simulink model "wattcredit_full_pcb_closedloop"  (R2023a)
settings: Solver=ode4  StartTime=0.0  StopTime=0.8  FixedStep=2e-5  RelTol=1e-3
libraries: simulink x3
settings Model: Creator=ruthm  LastModifiedBy=ruthm

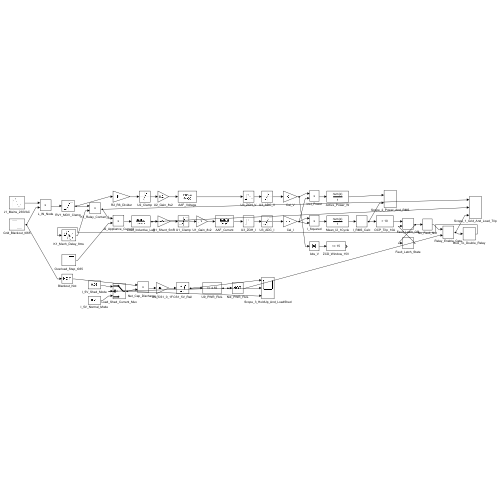
[thumbnail: Simulink's stored preview of the top-level diagram]
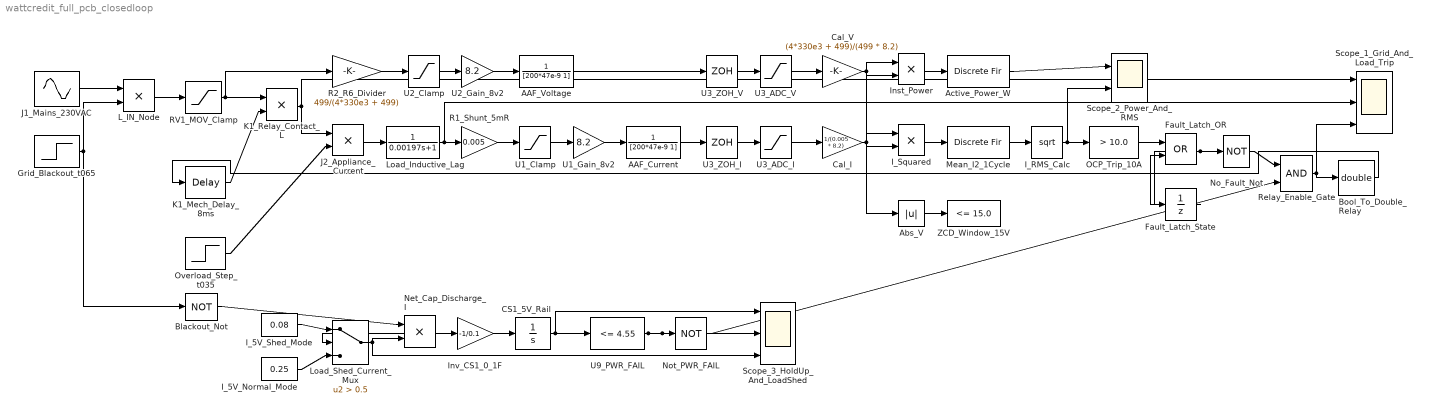
== system wattcredit_full_pcb_closedloop ==
  AAF_Current : TransferFcn  Denominator=[200*47e-9 1]
  AAF_Voltage : TransferFcn  Denominator=[200*47e-9 1]
  Abs_V : Abs  SaturateOnIntegerOverflow=off
  Active_Power_W : DiscreteFir  Coefficients=ones(1,80)/80  SampleTime=1/4000
  Blackout_Not : Logic  Operator=NOT  AllPortsSameDT=off  OutDataTypeStr=boolean
  Bool_To_Double_Relay : DataTypeConversion  OutDataTypeStr=double  SaturateOnIntegerOverflow=off  RndMeth=Floor
  CS1_5V_Rail : Integrator  InitialCondition=5.0  LimitOutput=on  UpperSaturationLimit=5.0  LowerSaturationLimit=0
  Cal_I : Gain  Gain=1/(0.005 * 8.2)
  Cal_V : Gain  Gain=(4*330e3 + 499)/(499 * 8.2)
  Fault_Latch_OR : Logic  Operator=OR  AllPortsSameDT=off  OutDataTypeStr=boolean
  Fault_Latch_State : UnitDelay  SampleTime=2e-5  HasFrameUpgradeWarning=on
  Grid_Blackout_t065 : Step  Time=0.65  Before=1  After=0  SampleTime=2e-5
  I_5V_Normal_Mode : Constant  Value=0.25
  I_5V_Shed_Mode : Constant  Value=0.08
  I_RMS_Calc : Sqrt
  I_Squared : Product
  Inst_Power : Product
  Inv_CS1_0_1F : Gain  Gain=-1/0.1
  J1_Mains_230VAC : Sin  Amplitude=230*sqrt(2)  Frequency=2*pi*50  SampleTime=2e-5
  J2_Appliance_Current : Product
  K1_Mech_Delay_8ms : TransportDelay  DelayTime=0.008  InitialOutput=1
  K1_Relay_Contact_L : Product
  L_IN_Node : Product
  Load_Inductive_Lag : TransferFcn  Denominator=[0.00197 1]
  Load_Shed_Current_Mux : Switch  Criteria=u2 > Threshold  Threshold=0.5  SaturateOnIntegerOverflow=off  InputSameDT=off
  Mean_I2_1Cycle : DiscreteFir  Coefficients=ones(1,80)/80  SampleTime=1/4000
  Net_Cap_Discharge_I : Product
  No_Fault_Not : Logic  Operator=NOT  AllPortsSameDT=off  OutDataTypeStr=boolean
  Not_PWR_FAIL : Logic  Operator=NOT  AllPortsSameDT=off  OutDataTypeStr=boolean
  OCP_Trip_10A : simulink/Logic and Bit Operations/Compare To Constant  relop=>  const=10.0  OutDataTypeStr=boolean
  Overload_Step_t035 : Step  Time=0.35  Before=5/230  After=12.5/230  SampleTime=2e-5
  R1_Shunt_5mR : Gain  Gain=0.005
  R2_R6_Divider : Gain  Gain=499/(4*330e3 + 499)
  RV1_MOV_Clamp : Saturate  UpperLimit=390  LowerLimit=-390
  Relay_Enable_Gate : Logic  AllPortsSameDT=off  OutDataTypeStr=boolean
  Scope_1_Grid_And_Load_Trip : Scope  NumInputPorts=3
  Scope_2_Power_And_RMS : Scope  NumInputPorts=2
  Scope_3_HoldUp_And_LoadShed : Scope  NumInputPorts=3
  U1_Clamp : Saturate  UpperLimit=0.25  LowerLimit=-0.25
  U1_Gain_8v2 : Gain  Gain=8.2
  U2_Clamp : Saturate  UpperLimit=0.25  LowerLimit=-0.25
  U2_Gain_8v2 : Gain  Gain=8.2
  U3_ADC_I : Saturate  UpperLimit=1.2  LowerLimit=-1.2
  U3_ADC_V : Saturate  UpperLimit=1.2  LowerLimit=-1.2
  U3_ZOH_I : ZeroOrderHold  SampleTime=1/4000
  U3_ZOH_V : ZeroOrderHold  SampleTime=1/4000
  U9_PWR_FAIL : simulink/Logic and Bit Operations/Compare To Constant  relop=<=  const=4.55  OutDataTypeStr=boolean
  ZCD_Window_15V : simulink/Logic and Bit Operations/Compare To Constant  relop=<=  const=15.0  OutDataTypeStr=boolean
  wires:
  J1_Mains_230VAC/1 -> L_IN_Node/1
  Grid_Blackout_t065/1 -> L_IN_Node/2, Blackout_Not/1
  L_IN_Node/1 -> RV1_MOV_Clamp/1
  RV1_MOV_Clamp/1 -> K1_Relay_Contact_L/1, R2_R6_Divider/1
  K1_Mech_Delay_8ms/1 -> K1_Relay_Contact_L/2
  K1_Relay_Contact_L/1 -> J2_Appliance_Current/1, Scope_1_Grid_And_Load_Trip/1
  Overload_Step_t035/1 -> J2_Appliance_Current/2
  J2_Appliance_Current/1 -> Load_Inductive_Lag/1
  R2_R6_Divider/1 -> U2_Clamp/1
  U2_Clamp/1 -> U2_Gain_8v2/1
  U2_Gain_8v2/1 -> AAF_Voltage/1
  AAF_Voltage/1 -> U3_ZOH_V/1
  U3_ZOH_V/1 -> U3_ADC_V/1
  U3_ADC_V/1 -> Cal_V/1
  Load_Inductive_Lag/1 -> R1_Shunt_5mR/1, Scope_1_Grid_And_Load_Trip/2
  R1_Shunt_5mR/1 -> U1_Clamp/1
  U1_Clamp/1 -> U1_Gain_8v2/1
  U1_Gain_8v2/1 -> AAF_Current/1
  AAF_Current/1 -> U3_ZOH_I/1
  U3_ZOH_I/1 -> U3_ADC_I/1
  U3_ADC_I/1 -> Cal_I/1
  Cal_V/1 -> Inst_Power/1, Abs_V/1
  Cal_I/1 -> Inst_Power/2, I_Squared/1, I_Squared/2
  Inst_Power/1 -> Active_Power_W/1
  Active_Power_W/1 -> Scope_2_Power_And_RMS/1
  I_Squared/1 -> Mean_I2_1Cycle/1
  Mean_I2_1Cycle/1 -> I_RMS_Calc/1
  I_RMS_Calc/1 -> Scope_2_Power_And_RMS/2, OCP_Trip_10A/1
  Abs_V/1 -> ZCD_Window_15V/1
  OCP_Trip_10A/1 -> Fault_Latch_OR/1
  Fault_Latch_OR/1 -> Fault_Latch_State/1, No_Fault_Not/1
  Fault_Latch_State/1 -> Fault_Latch_OR/2
  No_Fault_Not/1 -> Relay_Enable_Gate/1
  Not_PWR_FAIL/1 -> Relay_Enable_Gate/2
  Relay_Enable_Gate/1 -> Scope_1_Grid_And_Load_Trip/3, Bool_To_Double_Relay/1
  I_5V_Shed_Mode/1 -> Load_Shed_Current_Mux/1
  U9_PWR_FAIL/1 -> Not_PWR_FAIL/1, Scope_3_HoldUp_And_LoadShed/2, Load_Shed_Current_Mux/2
  I_5V_Normal_Mode/1 -> Load_Shed_Current_Mux/3
  Blackout_Not/1 -> Net_Cap_Discharge_I/1
  Load_Shed_Current_Mux/1 -> Net_Cap_Discharge_I/2, Scope_3_HoldUp_And_LoadShed/3
  Net_Cap_Discharge_I/1 -> Inv_CS1_0_1F/1
  Inv_CS1_0_1F/1 -> CS1_5V_Rail/1
  CS1_5V_Rail/1 -> U9_PWR_FAIL/1, Scope_3_HoldUp_And_LoadShed/1
  Bool_To_Double_Relay/1 -> K1_Mech_Delay_8ms/1
